simulink model "Deslaination_Simulation"  (R2026b)
settings: Solver=FixedStepDiscrete  StopTime=0  FixedStep=1
libraries: statsLibrary x1
settings Model: Creator=aashr_w74jbpz  LastModifiedBy=aashr_w74jbpz

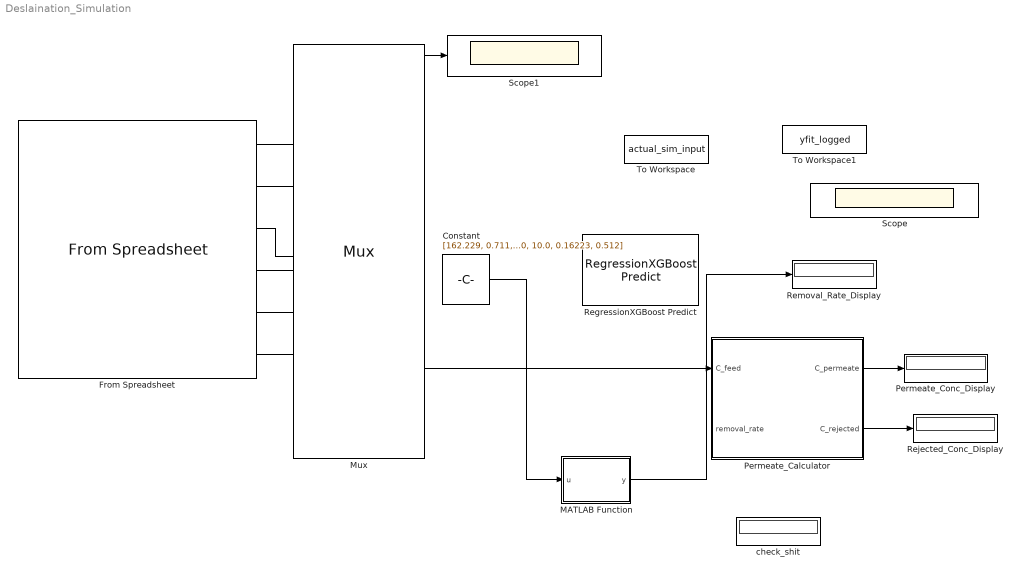
== system Deslaination_Simulation ==
  Constant : Constant  Value=[162.229, 0.711, 800.0, 10.0, 0.16223, 0.512]  VectorParams1D=off
  From Spreadsheet : FromSpreadsheet  FileName=\\wsl.localhost\ubuntu\home\aashr\-\Py\Minor_Spec\Papers\simulink_stream_data_6.xlsx  SheetName=DataStream  Range=A1:G1907  SampleTime=1
  MATLAB Function : MATLAB Function  TreatAsAtomicUnit=on
  Mux : Mux  Inputs=2
  Permeate_Calculator : MATLAB Function  TreatAsAtomicUnit=on
  Permeate_Conc_Display : Display
  RegressionXGBoost Predict : statsLibrary/Regression/RegressionXGBoost Predict  TrainedLearner=Mdl_v2  OutMin=[]  OutMax=[]  WeakLearnerOutMin=[]  WeakLearnerOutMax=[]
  Rejected_Conc_Display : Display
  Removal_Rate_Display : Display
  Scope : Scope
      settings: ActiveDisplayYMinimum=-5.47502227644463  ActiveDisplayYMaximum=110.48372931482982
  Scope1 : Scope
      settings: ActiveDisplayYMinimum=322.50000000000006  ActiveDisplayYMaximum=3297.5
  To Workspace : ToWorkspace  VariableName=actual_sim_input  SampleTime=-1
  To Workspace1 : ToWorkspace  VariableName=yfit_logged  SaveFormat=Timeseries  SampleTime=-1
  check_shit : Display
  wires:
  Permeate_Calculator/1(C_permeate) -> Permeate_Conc_Display/1
  Permeate_Calculator/2(C_rejected) -> Rejected_Conc_Display/1
  From Spreadsheet/1 -> ?
  From Spreadsheet/2 -> ?
  From Spreadsheet/5 -> Permeate_Calculator/1(C_feed)
  From Spreadsheet/6 -> ?
  From Spreadsheet/3 -> Scope1/1
  From Spreadsheet/4 -> ?
  Constant/1 -> MATLAB Function/1(u)
  MATLAB Function/1(y) -> Removal_Rate_Display/1

== matlab function Deslaination_Simulation/Permeate_Calculator ==
  data: C_feed input; C_permeate output; removal_rate input; C_rejected output
function [C_permeate, C_rejected] = Permeate_Calculator(C_feed, removal_rate)
%#codegen
% Clamp removal rate between 0% and 100%
rejection_frac = max(0.0, min(100.0, removal_rate)) / 100.0;

C_permeate = C_feed * (1.0 - rejection_frac);
C_rejected = C_feed * rejection_frac;
end

== matlab function Deslaination_Simulation/MATLAB Function ==
  data: u input; y output
function y = fcn(u)
coder.extrinsic('evalin');
coder.extrinsic('predict');
% Pre-assign output
y = 0.0;
% Ensure u is a 1x6 row vector regardless of input orientation
u_row = reshape(u, 1, 6);
% Fetch model from base workspace
mdl = evalin('base', 'Mdl_v2');
% Predict
y = double(predict(mdl, u_row));
end
